simulink model "BalanceCube_1D_Realistic"  (R2025b)
settings: Solver=daessc  StartTime=0.0  StopTime=12.0  MaxStep=0.005  RelTol=1e-4
values from neighbouring files (symbols this model uses):
  I_flywheel_kgm2 = 0.5 * m_web_kg * (r_in_eff^2) +                    0.5 * m_rim_kg * (flywheel_outer_radius_m^2 + r_in_eff^2)    [params_1d_cube.m]
  I_wheel_trans_kgm2 = 0.5 * I_wheel_spin_kgm2 + (1/12) * wheel_total_mass_kg * (flywheel_rim_thickness_m^2)    [params_1d_cube.m]
  L_center_m = square_side_m / sqrt(2) - pivot_corner_offset_m    [params_1d_cube.m]
  motor_Kt_NmA = motor_V_rated_V / w_noload_rads    [params_1d_cube.m]
  motor_stator_mass_kg = max(0.01, motor_mass_kg - motor_rotor_mass_kg)    [params_1d_cube.m]
  plate_mass_kg = plate_density_kgm3 * (square_side_m^2) * plate_thickness_m + extra_frame_mass_kg    [params_1d_cube.m]
  s = min(1.0, (t - 9.0) / 0.55)    [handAndKnockDisturbance.m]
  wheel_total_mass_kg = flywheel_mass_kg + motor_rotor_mass_kg    [params_1d_cube.m]
undefined symbols (not defined in the file or in its folder): com_imbalance_offset_m, gear_backlash_deg, motor_rotor_J_kgm2, plate_thickness_m, square_side_m, table_stop_deg, Ts_ctrl, X, Y, Z
libraries: sm_lib x11, fl_lib x9, nesl_utility x7, ee_lib x1
settings Model: Creator=thanotos  LastModifiedBy=thanotos

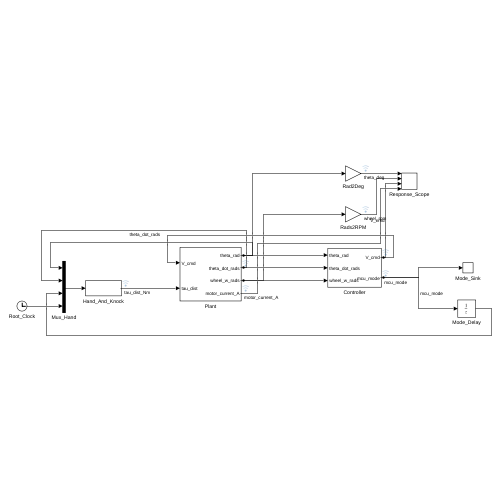
[thumbnail: Simulink's stored preview of the top-level diagram]
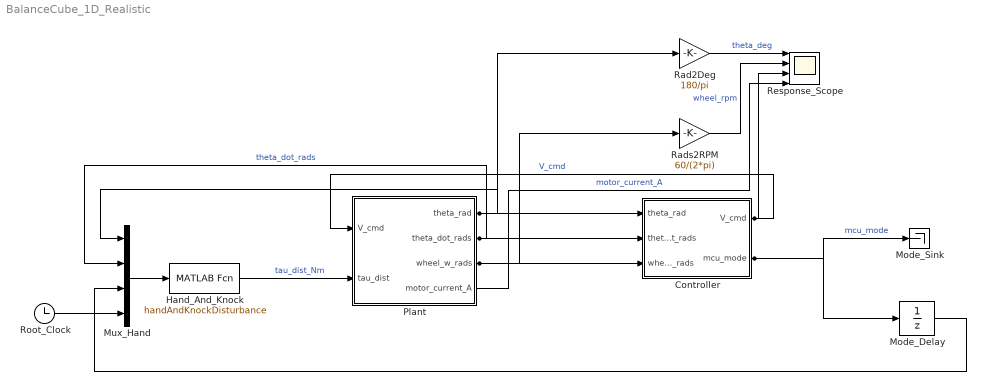
== system BalanceCube_1D_Realistic ==
  Controller : Subsystem
  Hand_And_Knock : MATLABFcn  MATLABFcn=handAndKnockDisturbance  OutputDimensions=1  SampleTime=0
  Mode_Delay : UnitDelay  SampleTime=Ts_ctrl  HasFrameUpgradeWarning=on
  Mode_Sink : Terminator
  Mux_Hand : Mux
  Plant : Subsystem
  Rad2Deg : Gain  Gain=180/pi
  Rads2RPM : Gain  Gain=60/(2*pi)
  Response_Scope : Scope  NumInputPorts=4
  Root_Clock : Clock
  wires:
  Hand_And_Knock/1 -> Plant/2(tau_dist)  "tau_dist_Nm"
  Mux_Hand/1 -> Hand_And_Knock/1
  Root_Clock/1 -> Mux_Hand/4
  Mode_Delay/1 -> Mux_Hand/3
  Controller/2(mcu_mode) -> Mode_Delay/1, Mode_Sink/1  "mcu_mode"
  Controller/1(V_cmd) -> Response_Scope/3, Plant/1(V_cmd)  "V_cmd"
  Plant/1(theta_rad) -> Controller/1(theta_rad), Rad2Deg/1, Mux_Hand/1
  Plant/2(theta_dot_rads) -> Mux_Hand/2, Controller/2(theta_dot_rads)  "theta_dot_rads"
  Plant/3(wheel_w_rads) -> Rads2RPM/1, Controller/3(wheel_w_rads)
  Rad2Deg/1 -> Response_Scope/1  "theta_deg"
  Rads2RPM/1 -> Response_Scope/2  "wheel_rpm"
  Plant/4(motor_current_A) -> Response_Scope/4  "motor_current_A"

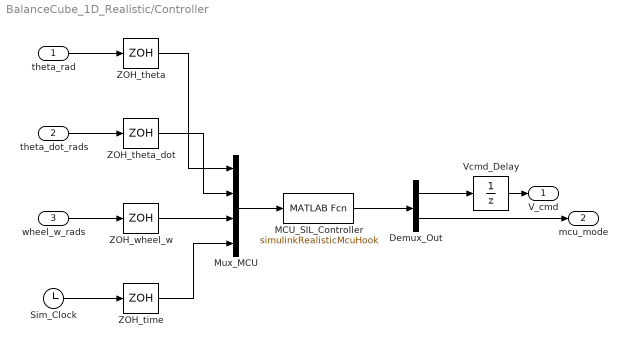
== system BalanceCube_1D_Realistic/Controller ==
  theta_rad : Inport
  theta_dot_rads : Inport  Port=2
  wheel_w_rads : Inport  Port=3
  Demux_Out : Demux  Outputs=2
  MCU_SIL_Controller : MATLABFcn  MATLABFcn=simulinkRealisticMcuHook  OutputDimensions=2  SampleTime=Ts_ctrl
  Mux_MCU : Mux
  Sim_Clock : Clock
  Vcmd_Delay : UnitDelay  SampleTime=Ts_ctrl  HasFrameUpgradeWarning=on
  ZOH_theta : ZeroOrderHold  SampleTime=Ts_ctrl
  ZOH_theta_dot : ZeroOrderHold  SampleTime=Ts_ctrl
  ZOH_time : ZeroOrderHold  SampleTime=Ts_ctrl
  ZOH_wheel_w : ZeroOrderHold  SampleTime=Ts_ctrl
  V_cmd : Outport
  mcu_mode : Outport  Port=2
  wires:
  Demux_Out/2 -> mcu_mode/1
  wheel_w_rads/1 -> ZOH_wheel_w/1
  theta_dot_rads/1 -> ZOH_theta_dot/1
  theta_rad/1 -> ZOH_theta/1
  ZOH_theta/1 -> Mux_MCU/1
  ZOH_theta_dot/1 -> Mux_MCU/2
  ZOH_wheel_w/1 -> Mux_MCU/3
  Sim_Clock/1 -> ZOH_time/1
  ZOH_time/1 -> Mux_MCU/4
  Mux_MCU/1 -> MCU_SIL_Controller/1
  MCU_SIL_Controller/1 -> Demux_Out/1
  Vcmd_Delay/1 -> V_cmd/1
  Demux_Out/1 -> Vcmd_Delay/1

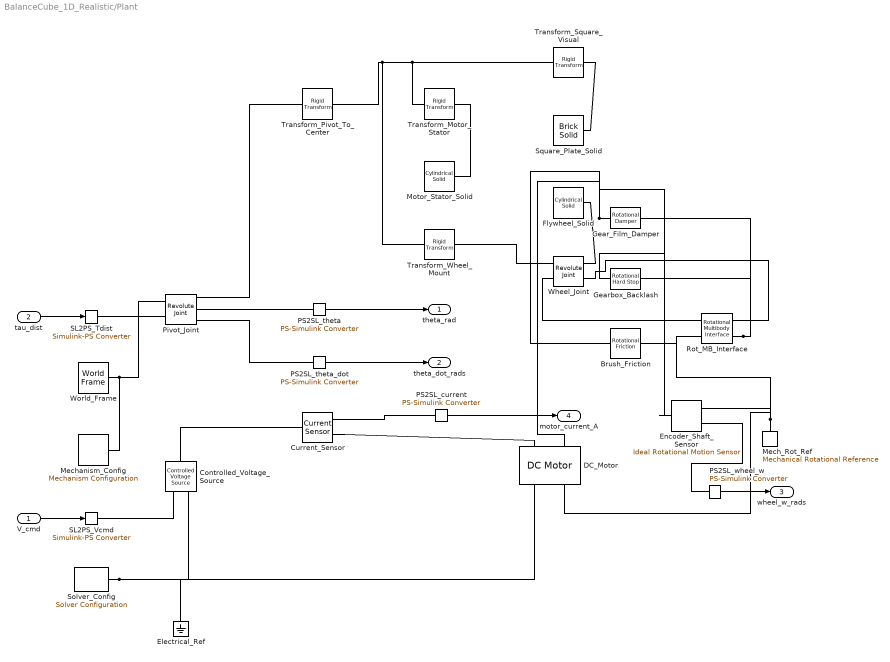
== system BalanceCube_1D_Realistic/Plant ==
  V_cmd : Inport
  tau_dist : Inport  Port=2
  Brush_Friction : fl_lib/Mechanical/Rotational Elements/Rotational Friction  brkwy_trq=motor_T_breakaway_Nm N*m  brkwy_vel=0.5 rad/s  Col_trq=motor_T_coulomb_Nm N*m  visc_coef=0 N*m*s/rad  w_specify=off  w_priority=None  w=0 rad/s  w_nominal_specify=off  w_nominal_value=1  w_nominal_unit=rad/s  t_specify=off  t_priority=None  t=0 N*m  t_nominal_specify=off  t_nominal_value=1  t_nominal_unit=N*m
  Controlled_Voltage_Source : fl_lib/Electrical/Electrical Sources/Controlled Voltage Source
  Current_Sensor : fl_lib/Electrical/Electrical Sensors/Current Sensor
  DC_Motor : ee_lib/Electromechanical/Brushed Motors/DC Motor  field_option=ee.enum.field_option.pm  Rf=100 Ohm  Lf=1 H  Laf=0.15 H  If0=0 A  parameterization=ee.enum.dcparam_option.circuit_param  Ra=motor_Ra_Ohm Ohm  La=motor_La_H H  emf_or_torque=ee.enum.emf_or_torque.ki  Kv=0.072e-3 V/rpm  Ki=motor_Kt_NmA N*m/A  T_stall=0.24e-3 N*m  w_max=19100 rpm  w_rated=15000 rpm  P_rated=0.08 W  V_rated=1.5 V  lam_param=ee.enum.lam_param.damping  i_noload=0 A  V_i_noload=1.5 V  J=motor_rotor_J_kgm2 kg*m^2  lam=motor_b_viscous_Nms N*m*s/rad  speed0=0 rpm  alpha=3.93e-3 1/K  Tmeas=25 degC  thermal_mass=100 J/K  initial_temperature=25 degC
  Electrical_Ref : fl_lib/Electrical/Electrical Elements/Electrical Reference
  Encoder_Shaft_Sensor : fl_lib/Mechanical/Mechanical Sensors/Ideal Rotational Motion Sensor  reference=foundation.enum.MeasurementReference.difference  acceleration_port=false  velocity_port=true  position_port=false  wrap_angle=off  offset=0 rad
      settings: InternalSimscapePortConfiguration="{\"Bottom\":[],\"Left\":[{\"id\":\"R\",\"label\":\"R\",\"type\":\"foundation.mechanical.rotational.rotational\"}],\"Right\":[{\"id\":\"C\",\"label\":\"C\",\"type\":\"foundation.mechanical.rotational.rotational\"},{\"id\":\"W\",\"label\":\"W\",\"type\":\"output\"}],\"Top\":[]}"
  Flywheel_Solid : sm_lib/Body Elements/Cylindrical Solid  CylinderRadius=flywheel_outer_radius_m  CylinderRadiusUnits=m  CylinderLength=flywheel_rim_thickness_m  CylinderLengthUnits=m  ExportEntireGeometry=off  InertiaType=Custom  BasedOnType=Mass  Density=1000  DensityUnits=kg/m^3  Mass=wheel_total_mass_kg  MassUnits=kg  CenterOfMass=[0 0 0]  CenterOfMassUnits=m  MomentsOfInertia=[I_wheel_trans_kgm2, I_wheel_trans_kgm2, I_flywheel_kgm2]  MomentsOfInertiaUnits=kg*m^2  ProductsOfInertia=[0 0 0]  ProductsOfInertiaUnits=kg*m^2  GraphicType=FromGeometry  MarkerShape=Sphere  MarkerSize=10  GraphicVisPropType=SimpleVisualProperties  GraphicDiffuseColor=[0.82 0.67 0.24]  GraphicOpacity=1  GraphicSpecularColor=[0.5 0.5 0.5 1.0]  GraphicAmbientColor=[0.15 0.15 0.15 1.0]  GraphicEmissiveColor=[0.0 0.0 0.0 1.0]  GraphicShininess=75  DoExposeReferenceFrame=on  SerializedFrames=<Frames/>
  Gear_Film_Damper : fl_lib/Mechanical/Rotational Elements/Rotational Damper  D=1e-4 N*m*s/rad  w_specify=off  w_priority=None  w=0 rad/s  w_nominal_specify=off  w_nominal_value=1  w_nominal_unit=rad/s  t_specify=off  t_priority=None  t=0 N*m  t_nominal_specify=off  t_nominal_value=1  t_nominal_unit=N*m
  Gearbox_Backlash : fl_lib/Mechanical/Rotational Elements/Rotational Hard Stop  upper_bnd=0.5*deg2rad(gear_backlash_deg) rad  lower_bnd=-0.5*deg2rad(gear_backlash_deg) rad  model=simscape.enum.hardstop.smooth  stiff_up=80 N*m/rad  stiff_low=80 N*m/rad  D_up=0.1 N*m*s/rad  D_low=0.1 N*m*s/rad  transition=0.001 rad  coeff_rest=0.7  w_tol=0.1 rad/s  trq_tol=0.001 N*m  w_specify=off  w_priority=None  w=0 rad/s  w_nominal_specify=off  w_nominal_value=1  w_nominal_unit=rad/s  t_specify=off  t_priority=None  t=0 N*m  t_nominal_specify=off  t_nominal_value=1  t_nominal_unit=N*m  phi_specify=off  phi_priority=High  phi=0 rad  phi_nominal_specify=off  phi_nominal_value=1  phi_nominal_unit=rad  M_specify=off  M_priority=None  M=0
  Mech_Rot_Ref : fl_lib/Mechanical/Rotational Elements/Mechanical Rotational Reference
  Mechanism_Config : sm_lib/Utilities/Mechanism Configuration  UniformGravity=Constant  GravityVector=[0 -9.80665 0]  GravityVectorUnits=m/s^2  LinearizationDelta=0.001  JointModeTransitionNonlinearIterations=2
  Motor_Stator_Solid : sm_lib/Body Elements/Cylindrical Solid  CylinderRadius=0.0185  CylinderRadiusUnits=m  CylinderLength=0.045  CylinderLengthUnits=m  ExportEntireGeometry=off  InertiaType=CalculateFromGeometry  BasedOnType=Mass  Density=1000  DensityUnits=kg/m^3  Mass=motor_stator_mass_kg  MassUnits=kg  CenterOfMass=[0 0 0]  CenterOfMassUnits=m  MomentsOfInertia=[1 1 1]  MomentsOfInertiaUnits=kg*m^2  ProductsOfInertia=[0 0 0]  ProductsOfInertiaUnits=kg*m^2  GraphicType=FromGeometry  MarkerShape=Sphere  MarkerSize=10  GraphicVisPropType=SimpleVisualProperties  GraphicDiffuseColor=[0.55 0.60 0.65]  GraphicOpacity=1  GraphicSpecularColor=[0.5 0.5 0.5 1.0]  GraphicAmbientColor=[0.15 0.15 0.15 1.0]  GraphicEmissiveColor=[0.0 0.0 0.0 1.0]  GraphicShininess=75  DoExposeReferenceFrame=on  SerializedFrames=<Frames/>
  PS2SL_current : nesl_utility/PS-Simulink Converter  PhysicalDomain=network_engine_domain  SubClassName=ps_output  LeftPortType=input  RightPortType=output  PseudoPeriodic=off  Frequencies=[]  VectorFormat=inherit  Unit=A  AffineConversion=off
  PS2SL_theta : nesl_utility/PS-Simulink Converter  PhysicalDomain=network_engine_domain  SubClassName=ps_output  LeftPortType=input  RightPortType=output  PseudoPeriodic=off  Frequencies=[]  VectorFormat=inherit  Unit=rad  AffineConversion=off
  PS2SL_theta_dot : nesl_utility/PS-Simulink Converter  PhysicalDomain=network_engine_domain  SubClassName=ps_output  LeftPortType=input  RightPortType=output  PseudoPeriodic=off  Frequencies=[]  VectorFormat=inherit  Unit=rad/s  AffineConversion=off
  PS2SL_wheel_w : nesl_utility/PS-Simulink Converter  PhysicalDomain=network_engine_domain  SubClassName=ps_output  LeftPortType=input  RightPortType=output  PseudoPeriodic=off  Frequencies=[]  VectorFormat=inherit  Unit=rad/s  AffineConversion=off
  Pivot_Joint : sm_lib/Joints/Revolute Joint  JointMode=Normal  CompositeWrenchDir=FollowerOnBase  CompositeWrenchFrame=BaseFrame  SenseConstraintForce=off  SenseConstraintTorque=off  SenseTotalForce=off  SenseTotalTorque=off  PositionTargetSpecify=on  PositionTargetPriority=High  PositionTargetValue=theta0_deg  PositionTargetValueUnits=deg  VelocityTargetSpecify=on  VelocityTargetPriority=High  VelocityTargetValue=0  VelocityTargetValueUnits=rad/s  EquilibriumPosition=0  EquilibriumPositionUnits=deg  SpringStiffness=0  SpringStiffnessUnits=N*m/deg  DampingCoefficient=b_pivot_Nms  DampingCoefficientUnits=N*m/(rad/s)  LowerLimitSpecify=on  LowerLimitBound=-table_stop_deg  LowerLimitBoundUnits=deg  LowerLimitStiffness=50  LowerLimitStiffnessUnits=N*m/deg  LowerLimitDamping=0.8  LowerLimitDampingUnits=N*m/(deg/s)  LowerLimitTransitionRegionWidth=0.5  LowerLimitTransitionRegionWidthUnits=deg  UpperLimitSpecify=on  UpperLimitBound=table_stop_deg  UpperLimitBoundUnits=deg  UpperLimitStiffness=50  UpperLimitStiffnessUnits=N*m/deg  UpperLimitDamping=0.8  UpperLimitDampingUnits=N*m/(deg/s)  UpperLimitTransitionRegionWidth=0.5  UpperLimitTransitionRegionWidthUnits=deg  TorqueActuationMode=InputTorque  MotionActuationMode=ComputedMotion  SensePosition=on  SenseVelocity=on  SenseAcceleration=off  SenseTorqueForce=off  SenseLowerLimitTorqueForce=off  SenseUpperLimitTorqueForce=off
  Rot_MB_Interface : fl_lib/Mechanical/Multibody Interfaces/Rotational Multibody Interface
  SL2PS_Tdist : nesl_utility/Simulink-PS Converter  PhysicalDomain=network_engine_domain  SubClassName=ps_input  LeftPortType=input  RightPortType=output  PseudoPeriodic=off  Frequencies=[]  NoiseDistribution=none  NoiseParameters=[]  Unit=N*m  AffineConversion=off  FilteringAndDerivatives=filter  SimscapeFilterOrder=1  InputFilterTimeConstant=0.0002  UdotUserProvided=0
  SL2PS_Vcmd : nesl_utility/Simulink-PS Converter  PhysicalDomain=network_engine_domain  SubClassName=ps_input  LeftPortType=input  RightPortType=output  PseudoPeriodic=off  Frequencies=[]  NoiseDistribution=none  NoiseParameters=[]  Unit=V  AffineConversion=off  FilteringAndDerivatives=filter  SimscapeFilterOrder=1  InputFilterTimeConstant=0.0002  UdotUserProvided=0
  Solver_Config : nesl_utility/Solver Configuration  PhysicalDomain=network_engine_domain  SubClassName=solver  LeftPortType=input  RightPortType=generic  Tones=[]  Harmonics=[]  SimulateNoise=off  Profile=off  UseLocalSampling=off  EnableSwitchedLinearOptims=on  FrequencyDomain=off  UseCCode=off  RelTol=0.001  AbsTol=0.001  MinStep=1e-09  ToWorkspace=off  RevertToSquareIcSolve=off  NumHomotopyIterations=100  PhasorMode=off  PhasorModeNumHarmonics=1  ConsistencySolver=NEWTON_XTOL_AFTER_FTOL  IndexReductionMethod=DerivativeReplacement  DoDC=off  ResidualTolerance=1e-09  ConsistencyTolSource=GLOBAL  ConsistencyAbsTol=0.001  ConsistencyRelTol=0.001  ConsistencyTolFactor=0.001  UseLocalSolver=off  LocalSolverChoice=NE_BACKWARD_EULER_ADVANCER  ResolveIndetEquations=on  FunctionEvalNumThread=1  LocalSolverSampleTime=0.001  DoFixedCost=off  MaxNonlinIter=3  MaxModeIter=2  ComputeImpulses=off  ImpulseIterations=2  LinearAlgebra=auto  LinearAlgebraNumThread=0  EquationFormulation=NE_TIME_EF  DelaysMemoryBudget=1024  AutomaticFiltering=on  FilteringTimeConstant=0.001  PartitionStorageMethod=AS_NEEDED  PartitionMemoryBudget=1024  PartitionMethod=ROBUST  MultibodyUseLocalSolver=off  MultibodyLocalSolverChoice=ODE1  MultibodyLocalSolverSampleTime=0.001
  Square_Plate_Solid : sm_lib/Body Elements/Brick Solid  BrickDimensions=[square_side_m, square_side_m, plate_thickness_m]  BrickDimensionsUnits=m  ExportEntireGeometry=off  InertiaType=CalculateFromGeometry  BasedOnType=Mass  Density=1000  DensityUnits=kg/m^3  Mass=plate_mass_kg  MassUnits=kg  CenterOfMass=[0 0 0]  CenterOfMassUnits=m  MomentsOfInertia=[1 1 1]  MomentsOfInertiaUnits=kg*m^2  ProductsOfInertia=[0 0 0]  ProductsOfInertiaUnits=kg*m^2  GraphicType=FromGeometry  MarkerShape=Sphere  MarkerSize=10  GraphicVisPropType=SimpleVisualProperties  GraphicDiffuseColor=[0.75 0.88 0.95]  GraphicOpacity=0.55  GraphicSpecularColor=[0.5 0.5 0.5 1.0]  GraphicAmbientColor=[0.15 0.15 0.15 1.0]  GraphicEmissiveColor=[0.0 0.0 0.0 1.0]  GraphicShininess=75  DoExposeReferenceFrame=on  SerializedFrames=<Frames/>
  Transform_Motor_Stator : sm_lib/Frames and Transforms/Rigid Transform  RotationMethod=None  FollAlignAxisA=+X  BaseAlignAxisA=+Y  FollAlignAxisB=+Y  BaseAlignAxisB=+Z  RotationStandardAxis=+Z  RotationAngle=0  RotationAngleUnits=deg  RotationArbitraryAxis=[0 0 1]  RotationSequenceAxes=FollowerAxes  RotationSequence=XYX  RotationSequenceAngles=[0 0 0]  RotationSequenceAnglesUnits=deg  RotationMatrix=[1 0 0;0 1 0;0 0 1]  Quaternion=[1 0 0 0]  TranslationMethod=StandardAxis  TranslationCartesianOffset=[0 0 0]  TranslationCartesianOffsetUnits=m  TranslationStandardAxis=-Z  TranslationStandardOffset=0.025  TranslationStandardOffsetUnits=m  TranslationROffset=0  TranslationROffsetUnits=m  TranslationThetaOffset=0  TranslationThetaOffsetUnits=deg  TranslationZOffset=0  TranslationZOffsetUnits=m
  Transform_Pivot_To_Center : sm_lib/Frames and Transforms/Rigid Transform  RotationMethod=None  FollAlignAxisA=+X  BaseAlignAxisA=+Y  FollAlignAxisB=+Y  BaseAlignAxisB=+Z  RotationStandardAxis=+Z  RotationAngle=0  RotationAngleUnits=deg  RotationArbitraryAxis=[0 0 1]  RotationSequenceAxes=FollowerAxes  RotationSequence=XYX  RotationSequenceAngles=[0 0 0]  RotationSequenceAnglesUnits=deg  RotationMatrix=[1 0 0;0 1 0;0 0 1]  Quaternion=[1 0 0 0]  TranslationMethod=Cartesian  TranslationCartesianOffset=[com_imbalance_offset_m, L_center_m, 0]  TranslationCartesianOffsetUnits=m  TranslationStandardAxis=+Z  TranslationStandardOffset=0  TranslationStandardOffsetUnits=m  TranslationROffset=0  TranslationROffsetUnits=m  TranslationThetaOffset=0  TranslationThetaOffsetUnits=deg  TranslationZOffset=0  TranslationZOffsetUnits=m
  Transform_Square_Visual : sm_lib/Frames and Transforms/Rigid Transform  RotationMethod=StandardAxis  FollAlignAxisA=+X  BaseAlignAxisA=+Y  FollAlignAxisB=+Y  BaseAlignAxisB=+Z  RotationStandardAxis=+Z  RotationAngle=45  RotationAngleUnits=deg  RotationArbitraryAxis=[0 0 1]  RotationSequenceAxes=FollowerAxes  RotationSequence=XYX  RotationSequenceAngles=[0 0 0]  RotationSequenceAnglesUnits=deg  RotationMatrix=[1 0 0;0 1 0;0 0 1]  Quaternion=[1 0 0 0]  TranslationMethod=None  TranslationCartesianOffset=[0 0 0]  TranslationCartesianOffsetUnits=m  TranslationStandardAxis=+Z  TranslationStandardOffset=0  TranslationStandardOffsetUnits=m  TranslationROffset=0  TranslationROffsetUnits=m  TranslationThetaOffset=0  TranslationThetaOffsetUnits=deg  TranslationZOffset=0  TranslationZOffsetUnits=m
  Transform_Wheel_Mount : sm_lib/Frames and Transforms/Rigid Transform  RotationMethod=None  FollAlignAxisA=+X  BaseAlignAxisA=+Y  FollAlignAxisB=+Y  BaseAlignAxisB=+Z  RotationStandardAxis=+Z  RotationAngle=0  RotationAngleUnits=deg  RotationArbitraryAxis=[0 0 1]  RotationSequenceAxes=FollowerAxes  RotationSequence=XYX  RotationSequenceAngles=[0 0 0]  RotationSequenceAnglesUnits=deg  RotationMatrix=[1 0 0;0 1 0;0 0 1]  Quaternion=[1 0 0 0]  TranslationMethod=StandardAxis  TranslationCartesianOffset=[0 0 0]  TranslationCartesianOffsetUnits=m  TranslationStandardAxis=+Z  TranslationStandardOffset=0.015  TranslationStandardOffsetUnits=m  TranslationROffset=0  TranslationROffsetUnits=m  TranslationThetaOffset=0  TranslationThetaOffsetUnits=deg  TranslationZOffset=0  TranslationZOffsetUnits=m
  Wheel_Joint : sm_lib/Joints/Revolute Joint  JointMode=Normal  CompositeWrenchDir=FollowerOnBase  CompositeWrenchFrame=BaseFrame  SenseConstraintForce=off  SenseConstraintTorque=off  SenseTotalForce=off  SenseTotalTorque=off  PositionTargetSpecify=on  PositionTargetPriority=Low  PositionTargetValue=0  PositionTargetValueUnits=deg  VelocityTargetSpecify=on  VelocityTargetPriority=High  VelocityTargetValue=0  VelocityTargetValueUnits=rad/s  EquilibriumPosition=0  EquilibriumPositionUnits=deg  SpringStiffness=0  SpringStiffnessUnits=N*m/deg  DampingCoefficient=0  DampingCoefficientUnits=N*m/(rad/s)  LowerLimitSpecify=off  LowerLimitBound=-90  LowerLimitBoundUnits=deg  LowerLimitStiffness=1e4  LowerLimitStiffnessUnits=N*m/deg  LowerLimitDamping=10  LowerLimitDampingUnits=N*m/(deg/s)  LowerLimitTransitionRegionWidth=0.1  LowerLimitTransitionRegionWidthUnits=deg  UpperLimitSpecify=off  UpperLimitBound=90  UpperLimitBoundUnits=deg  UpperLimitStiffness=1e4  UpperLimitStiffnessUnits=N*m/deg  UpperLimitDamping=10  UpperLimitDampingUnits=N*m/(deg/s)  UpperLimitTransitionRegionWidth=0.1  UpperLimitTransitionRegionWidthUnits=deg  TorqueActuationMode=InputTorque  MotionActuationMode=ComputedMotion  SensePosition=off  SenseVelocity=on  SenseAcceleration=off  SenseTorqueForce=off  SenseLowerLimitTorqueForce=off  SenseUpperLimitTorqueForce=off
  World_Frame : sm_lib/Frames and Transforms/World Frame
  theta_rad : Outport
  theta_dot_rads : Outport  Port=2
  wheel_w_rads : Outport  Port=3
  motor_current_A : Outport  Port=4
  wires:
  PS2SL_current/1 -> motor_current_A/1
  PS2SL_theta_dot/1 -> theta_dot_rads/1
  PS2SL_theta/1 -> theta_rad/1
  tau_dist/1 -> SL2PS_Tdist/1
  V_cmd/1 -> SL2PS_Vcmd/1
  PS2SL_wheel_w/1 -> wheel_w_rads/1
  connections:
  Current_Sensor/RConn1 -- PS2SL_current/LConn1
  Controlled_Voltage_Source/LConn1 -- Current_Sensor/LConn1
  SL2PS_Vcmd/RConn1 -- Controlled_Voltage_Source/RConn1
  Wheel_Joint/RConn1 -- Flywheel_Solid/RConn1
  Transform_Wheel_Mount/RConn1 -- Wheel_Joint/LConn1
  Transform_Motor_Stator/RConn1 -- Motor_Stator_Solid/RConn1
  Transform_Square_Visual/RConn1 -- Square_Plate_Solid/RConn1
  Transform_Pivot_To_Center/RConn1 -- Transform_Square_Visual/LConn1 -- Transform_Motor_Stator/LConn1 -- Transform_Wheel_Mount/LConn1
  Pivot_Joint/RConn3 -- PS2SL_theta_dot/LConn1
  Pivot_Joint/RConn2 -- PS2SL_theta/LConn1
  Pivot_Joint/RConn1 -- Transform_Pivot_To_Center/LConn1
  SL2PS_Tdist/RConn1 -- Pivot_Joint/LConn2
  Pivot_Joint/LConn1 -- World_Frame/RConn1 -- Mechanism_Config/RConn1
  Encoder_Shaft_Sensor/RConn2 -- PS2SL_wheel_w/LConn1
  Gearbox_Backlash/RConn1 -- Gear_Film_Damper/RConn1 -- Rot_MB_Interface/RConn2
  Encoder_Shaft_Sensor/LConn1 -- DC_Motor/LConn2 -- Gear_Film_Damper/LConn1 -- Gearbox_Backlash/LConn1 -- Brush_Friction/LConn1
  Wheel_Joint/RConn2 -- Rot_MB_Interface/RConn1
  Controlled_Voltage_Source/RConn2 -- Solver_Config/RConn1 -- DC_Motor/RConn1 -- Electrical_Ref/LConn1
  Current_Sensor/RConn2 -- DC_Motor/LConn1
  Mech_Rot_Ref/LConn1 -- Encoder_Shaft_Sensor/RConn1 -- Brush_Friction/RConn1 -- Rot_MB_Interface/LConn2 -- DC_Motor/RConn2
  Rot_MB_Interface/LConn1 -- Wheel_Joint/LConn2
